simulink model "StampFly_StudentBlocks"  (R2026b)
settings: Solver=VariableStepAuto
undefined symbols (not defined in the file): Bottom, Official
(part 6 of 6)

== stateflow chart StampFly_StudentBlocks/FlightSequence/OfficialTakeoffHover400/SensorProcessing400/AltitudeKalman ==
  note: 高度Kalman：状態=[鉛直速度;高度;加速度バイアス]。400 Hzで最新保持ToFと鉛直加速度を使用。公式resetは内部推定xを保持。
  state Calculate
    en: [height,velocity,bias]=stepFn(alt,az,mode,dt,parkingReset);
    du: [height,velocity,bias]=stepFn(alt,az,mode,dt,parkingReset);
  (default) -> Calculate
  data: alt function_input; az function_input; mode function_input; dt function_input; parkingReset function_input; height function_output; velocity function_output; bias function_output; alt input single; az input single; mode input uint8; dt input single; parkingReset input boolean; height output single; velocity output single; bias output single
  function [height,velocity,bias]=stepFn(alt,az,mode,dt,parkingReset):
    | function [height,velocity,bias]=stepFn(alt,az,mode,dt,parkingReset)
    | % 日本語の説明はブロック注釈とDescriptionを参照。
    | %#codegen
    | persistent State First PreviousMode;
    | if isempty(State)
    | State=kalmanInitial();
    | First=false;
    | PreviousMode=uint8(0);
    | end
    |             if parkingReset,[~,State]=kalmanStep(single(0),single(0),dt,true,State);end
    |             if mode==3 && mode~=PreviousMode,First=false;end
    |             if mode>1
    |                 if First,[~,State]=kalmanStep(alt,az,dt,false,State);else,First=true;end
    |             end
    |             velocity=State.output(1);height=State.output(2);bias=State.output(3);PreviousMode=mode;
    | end
    | 
    | function [y,s] = kalmanStep(z,acc,h,resetState,s)
    | %KALMANSTEP Direct translation of Alt_kalman::update, state [v;z;bias].
    | % Preserve reset(): covariance and public output reset, private x is retained.
    | %#codegen
    | if resetState
    |     s.P = single(100)*eye(3,'single'); s.output(:) = single(0);
    | else
    |     p=s.P; b=single(-0.01); f=single(1)+h*b;
    |     xp=[s.x(1)+(acc-s.x(3))*h;s.x(2)+s.x(1)*h;s.x(3)*f];
    |     pp=zeros(3,3,'single');
    |     pp(1,1)=p(1,1)-h*(p(3,1)+p(1,3))+h*h*p(3,3)+h*h*single(0.01);
    |     pp(1,2)=h*(p(1,1)-p(3,2))-h*h*p(3,1)+p(1,2);
    |     pp(1,3)=f*(p(1,3)-h*p(3,3));
    |     pp(2,1)=h*(p(1,1)-p(2,3))-h*h*p(1,3)+p(2,1);
    |     pp(2,2)=h*h*p(1,1)+h*(p(2,1)+p(1,2))+p(2,2);
    |     pp(2,3)=f*(p(2,3)+h*p(1,3));
    |     pp(3,1)=f*(p(3,1)-h*p(3,3));
    |     pp(3,2)=f*(p(3,2)+h*p(3,1));
    |     pp(3,3)=f*f*p(3,3)+h*h;
    |     k=[pp(1,2);pp(2,2);pp(3,2)]/(pp(2,2)+single(0.004*0.004));
    |     e=z-xp(2); s.x=xp+k*e; s.output=s.x;
    |     s.P(1,:)=pp(1,:)-k(1)*pp(2,:);
    |     s.P(2,:)=pp(2,:)*(single(1)-k(2));
    |     s.P(3,:)=-k(3)*pp(2,:)+pp(3,:);
    | end
    | y=s.output;
    | end
    | 
    | function s = kalmanInitial()
    | %#codegen
    | s = struct('x',zeros(3,1,'single'),'P',single(100)*eye(3,'single'), ...
    |     'output',zeros(3,1,'single'));
    | end

== stateflow chart StampFly_StudentBlocks/FlightSequence/OfficialTakeoffHover400/SensorProcessing400/IMUAxisConversion ==
  note: IMU軸変換：センサーX/Yを入れ替えZの符号を反転。公式の加速度単位gを保持します。
  state Calculate
    en: [a,g]=stepFn(accelMps2,gyroRps);
    du: [a,g]=stepFn(accelMps2,gyroRps);
  (default) -> Calculate
  data: accelMps2 function_input; gyroRps function_input; a function_output; g function_output; accelMps2 input single; gyroRps input single; a output single; g output single
  function [a,g]=stepFn(accelMps2,gyroRps):
    | function [a,g]=stepFn(accelMps2,gyroRps)
    | % 日本語の説明はブロック注釈とDescriptionを参照。
    | %#codegen
    |             a=accelMps2([2 1 3])/single(9.80665);a(3)=-a(3);
    |             g=gyroRps([2 1 3]);g(3)=-g(3);
    | end

== stateflow chart StampFly_StudentBlocks/FlightSequence/OfficialTakeoffHover400/SensorProcessing400/IMUBiasCalibration ==
  note: 800周期の平均校正：ジャイロXYZと加速度Zのオフセットを平均します。400 Hzなので公称2秒です。
  state Calculate
    en: [offset,count]=stepFn(a,g,mode);
    du: [offset,count]=stepFn(a,g,mode);
  (default) -> Calculate
  data: a function_input; g function_input; mode function_input; offset function_output; count function_output; a input single; g input single; mode input uint8; offset output single; count output uint16
  function [offset,count]=stepFn(a,g,mode):
    | function [offset,count]=stepFn(a,g,mode)
    | % 日本語の説明はブロック注釈とDescriptionを参照。
    | %#codegen
    | persistent Offset Count;
    | if isempty(Offset)
    | Offset=zeros(4,1,'single');
    | Count=uint16(0);
    | end
    |             if mode==0,Offset(:)=single(0);Count=uint16(0);
    |             elseif mode==1 && Count<uint16(800)
    |                 n=single(Count);Offset=(n*Offset+[g;a(3)])/(n+single(1));Count=Count+uint16(1);
    |             end
    |             offset=Offset;count=Count;
    | end

== stateflow chart StampFly_StudentBlocks/FlightSequence/OfficialTakeoffHover400/SensorProcessing400/IMUFiltering ==
  note: IMUフィルター：加速度とジャイロは時定数3 ms、鉛直差分は100 ms。PARKING移行で状態をリセット。
  state Calculate
    en: [af,gf,azd]=stepFn(a,g,offset,mode,dt);
    du: [af,gf,azd]=stepFn(a,g,offset,mode,dt);
  (default) -> Calculate
  data: a function_input; g function_input; offset function_input; mode function_input; dt function_input; af function_output; gf function_output; azd function_output; a input single; g input single; offset input single; mode input uint8; dt input single; af output single; gf output single; azd output single
  function [af,gf,azd]=stepFn(a,g,offset,mode,dt):
    | function [af,gf,azd]=stepFn(a,g,offset,mode,dt)
    | % 日本語の説明はブロック注釈とDescriptionを参照。
    | %#codegen
    | persistent Filter Accel Gyro Azd PreviousMode;
    | if isempty(Filter)
    | Filter=zeros(7,1,'single');
    | Accel=zeros(3,1,'single');
    | Gyro=zeros(3,1,'single');
    | Azd=single(0);
    | PreviousMode=uint8(0);
    | end
    |             if mode==3 && mode~=PreviousMode,Filter(:)=single(0);end
    |             if mode>1
    |                 for j=1:3
    |                     Filter(j)=filterStep(a(j),dt,single(0.003),Filter(j));
    |                     Filter(j+3)=filterStep(g(j)-offset(j),dt,single(0.003),Filter(j+3));
    |                 end
    |                 Filter(7)=filterStep(a(3)-offset(4),dt,single(0.1),Filter(7));
    |                 Accel=Filter(1:3);Gyro=Filter(4:6);Azd=Filter(7);
    |             end
    |             af=Accel;gf=Gyro;azd=Azd;PreviousMode=mode;
    | end
    | 
    | function s = filterStep(u,h,T,s)
    | %FILTERSTEP Exact Filter::update, including operation ordering.
    | %#codegen
    | s = s*T/(T+h) + u*h/(T+h);
    | end

== stateflow chart StampFly_StudentBlocks/FlightSequence/OfficialTakeoffHover400/SensorProcessing400/MadgwickAttitude ==
  note: Madgwick姿勢推定：400 Hz、β=0.1。公式の高速逆平方根、軸の対応、Yaw+180°を保持。数式はこのChart内にあります。
  state Calculate
    en: [a,q]=stepFn(rates,accel,mode,reset);
    du: [a,q]=stepFn(rates,accel,mode,reset);
  (default) -> Calculate
  data: arg_rates function_input; arg_accel function_input; arg_mode function_input; arg_reset function_input; arg_a function_output; arg_q function_output; rates input single; accel input single; mode input uint8; reset input boolean; a output single; q output single
  function [arg_a,arg_q]=stepFn(arg_rates,arg_accel,arg_mode,arg_reset):
    | function [arg_a,arg_q]=stepFn(arg_rates,arg_accel,arg_mode,arg_reset)
    | % 日本語の説明はブロック注釈とDescriptionを参照。
    | %#codegen
    | persistent Q Angles;
    | if isempty(Q)
    | Q=single([1;0;0;0]);
    | Angles=zeros(3,1,'single');
    | end
    |             if arg_reset,Q=single([1;0;0;0]);end
    |             if arg_mode>1,[Angles,Q]=madgwickStep(arg_rates,arg_accel,Q,false);end
    |             arg_a=Angles;arg_q=Q;
    | end
    | 
    | function [attitude,arg_q] = madgwickStep(arg_rates,arg_accel,arg_q,arg_reset)
    | %MADGWICKSTEP Official updateIMU with body-axis conventions and invSqrt.
    | % Rates rad/s and arg_accel g in official body frame [forward;left;down].
    | % Madgwick is fixed 400 Hz even though other official filters use measured dt.
    | % Translation of lib/MdgwickAHRS/MadgwickAHRS.cpp; original license retained.
    | %#codegen
    | if arg_reset, arg_q=single([1;0;0;0]); end
    | q0=arg_q(1);q1=arg_q(2);q2=arg_q(3);q3=arg_q(4);
    | % Retain original rad->deg->rad conversion coefficients, including rounding.
    | g=arg_rates([2 1 3])*single(180/pi);g(3)=-g(3);
    | g=g*single(0.0174533);gx=g(1);gy=g(2);gz=g(3);
    | arg_a=arg_accel([2 1 3]);arg_a(3)=-arg_a(3);ax=arg_a(1);ay=arg_a(2);az=arg_a(3);
    | dq=single(0.5)*[-q1*gx-q2*gy-q3*gz; q0*gx+q2*gz-q3*gy; ...
    |     q0*gy-q1*gz+q3*gx; q0*gz+q1*gy-q2*gx];
    | if ax~=0 || ay~=0 || az~=0
    |     reciprocal=fastInvSqrt(ax*ax+ay*ay+az*az);
    |     ax=ax*reciprocal;ay=ay*reciprocal;az=az*reciprocal;
    |     q02=q0*q0;q12=q1*q1;q22=q2*q2;q32=q3*q3;
    |     q0x2=single(2)*q0;q1x2=single(2)*q1;q2x2=single(2)*q2;q3x2=single(2)*q3;
    |     q0x4=single(4)*q0;q1x4=single(4)*q1;q2x4=single(4)*q2;
    |     q1x8=single(8)*q1;q2x8=single(8)*q2;
    |     gradient=[q0x4*q22+q2x2*ax+q0x4*q12-q1x2*ay; ...
    |         q1x4*q32-q3x2*ax+single(4)*q02*q1-q0x2*ay-q1x4+q1x8*q12+q1x8*q22+q1x4*az; ...
    |         single(4)*q02*q2+q0x2*ax+q2x4*q32-q3x2*ay-q2x4+q2x8*q12+q2x8*q22+q2x4*az; ...
    |         single(4)*q12*q3-q1x2*ax+single(4)*q22*q3-q2x2*ay];
    |     reciprocal=fastInvSqrt(gradient(1)*gradient(1)+gradient(2)*gradient(2)+gradient(3)*gradient(3)+gradient(4)*gradient(4));
    |     gradient=gradient*reciprocal;
    |     dq=dq-single(0.1)*gradient;
    | end
    | arg_q=arg_q+dq*single(1/400);
    | reciprocal=fastInvSqrt(arg_q(1)*arg_q(1)+arg_q(2)*arg_q(2)+arg_q(3)*arg_q(3)+arg_q(4)*arg_q(4));arg_q=arg_q*reciprocal;
    | roll=atan2(arg_q(1)*arg_q(2)+arg_q(3)*arg_q(4),single(0.5)-arg_q(2)*arg_q(2)-arg_q(3)*arg_q(3));
    | pitch=asin(-single(2)*(arg_q(2)*arg_q(4)-arg_q(1)*arg_q(3)));
    | yaw=atan2(arg_q(2)*arg_q(3)+arg_q(1)*arg_q(4),single(0.5)-arg_q(3)*arg_q(3)-arg_q(4)*arg_q(4));
    | % Original getYaw adds 180 degrees; do not hide this offset.
    | attitude=[pitch*single(57.29578);roll*single(57.29578); ...
    |     -(yaw*single(57.29578)+single(180))]*single(pi/180);
    | end
    | 
    | function y=fastInvSqrt(x)
    | i=typecast(x,'uint32');i=uint32(hex2dec('5f3759df'))-bitshift(i,-1);
    | y=typecast(i,'single');half=single(0.5)*x;
    | y=y*(single(1.5)-half*y*y);y=y*(single(1.5)-half*y*y);
    | end

== stateflow chart StampFly_StudentBlocks/FlightSequence/OfficialTakeoffHover400/SensorProcessing400/SensorDiagnosticPack ==
  state Calculate
    en: [diag]=stepFn(az,bias,alt,offset,count);
    du: [diag]=stepFn(az,bias,alt,offset,count);
  (default) -> Calculate
  data: az function_input; bias function_input; alt function_input; offset function_input; count function_input; diag function_output; az input single; bias input single; alt input single; offset input single; count input uint16; diag output single
  function diag =stepFn(az,bias,alt,offset,count):
    | function diag =stepFn(az,bias,alt,offset,count)
    | % 日本語の説明はブロック注釈とDescriptionを参照。
    | %#codegen
    |             diag=[az;bias;alt;offset;single(count)];
    | end

== stateflow chart StampFly_StudentBlocks/Estimation/IMUFiltering ==
  note: IMUフィルター：加速度とジャイロは時定数3 ms、鉛直差分は100 ms。PARKING移行で状態をリセット。
  state Calculate
    en: [af,gf,azd]=stepFn(a,g,offset,mode,dt);
    du: [af,gf,azd]=stepFn(a,g,offset,mode,dt);
  (default) -> Calculate
  data: a function_input; g function_input; offset function_input; mode function_input; dt function_input; af function_output; gf function_output; azd function_output; a input single; g input single; offset input single; mode input uint8; dt input single; af output single; gf output single; azd output single
  function [af,gf,azd]=stepFn(a,g,offset,mode,dt):
    | function [af,gf,azd]=stepFn(a,g,offset,mode,dt)
    | % 日本語の説明はブロック注釈とDescriptionを参照。
    | %#codegen
    | persistent Filter Accel Gyro Azd PreviousMode;
    | if isempty(Filter)
    | Filter=zeros(7,1,'single');
    | Accel=zeros(3,1,'single');
    | Gyro=zeros(3,1,'single');
    | Azd=single(0);
    | PreviousMode=uint8(0);
    | end
    |             if mode==3 && mode~=PreviousMode,Filter(:)=single(0);end
    |             if mode>1
    |                 for j=1:3
    |                     Filter(j)=filterStep(a(j),dt,single(0.003),Filter(j));
    |                     Filter(j+3)=filterStep(g(j)-offset(j),dt,single(0.003),Filter(j+3));
    |                 end
    |                 Filter(7)=filterStep(a(3)-offset(4),dt,single(0.1),Filter(7));
    |                 Accel=Filter(1:3);Gyro=Filter(4:6);Azd=Filter(7);
    |             end
    |             af=Accel;gf=Gyro;azd=Azd;PreviousMode=mode;
    | end
    | 
    | function s = filterStep(u,h,T,s)
    | %FILTERSTEP Exact Filter::update, including operation ordering.
    | %#codegen
    | s = s*T/(T+h) + u*h/(T+h);
    | end

== stateflow chart StampFly_StudentBlocks/FlightSequence/OfficialTakeoffHover400/SensorProcessing400/SensorFlags ==
  note: フラグ判定：OverG、距離無効/高度上限、低電圧100回。PID制御や状態遷移で使います。
  state Calculate
    en: [flags]=stepFn(accel,azd,voltage,mode,altFlag,height,rawRange,dt,parkingReset,flipFlag);
    du: [flags]=stepFn(accel,azd,voltage,mode,altFlag,height,rawRange,dt,parkingReset,flipFlag);
  (default) -> Calculate
  data: arg_accel function_input; arg_azd function_input; arg_voltage function_input; arg_mode function_input; arg_altFlag function_input; arg_height function_input; arg_rawRange function_input; arg_dt function_input; arg_parkingReset function_input; arg_flags function_output; arg_flipFlag function_input; accel input single; azd input single; voltage input single; mode input uint8; altFlag input uint8; height input single; rawRange input int16; dt input single; parkingReset input boolean; flags output uint8; flipFlag input uint8
  function arg_flags =stepFn(arg_accel,arg_azd,arg_voltage,arg_mode,arg_altFlag,arg_height,arg_rawRange,arg_dt,arg_parkingReset,arg_flipFlag):
    | function arg_flags =stepFn(arg_accel,arg_azd,arg_voltage,arg_mode,arg_altFlag,arg_height,arg_rawRange,arg_dt,arg_parkingReset,arg_flipFlag)
    | % 日本語の説明はブロック注釈とDescriptionを参照。
    | %#codegen
    | persistent Norm Voltage OverG RangeFlag LowVoltage PreviousMode;
    | if isempty(Norm)
    | Norm=single(0);
    | Voltage=single(0);
    | OverG=uint8(0);
    | RangeFlag=uint8(0);
    | LowVoltage=uint8(0);
    | PreviousMode=uint8(0);
    | end
    |             if arg_parkingReset,OverG=uint8(0);RangeFlag=uint8(0);end
    |             if arg_mode==3 && arg_mode~=PreviousMode,Norm=single(0);end
    |             if arg_mode>1
    |                 if (arg_height>single(2) && arg_altFlag~=0 && arg_flipFlag==0) || arg_rawRange==0,RangeFlag=min(RangeFlag+uint8(1),uint8(20));else,RangeFlag=uint8(0);end
    |             end
    |             normA=sqrt(arg_accel(1)*arg_accel(1)+arg_accel(2)*arg_accel(2)+arg_azd*arg_azd);
    |             Norm=filterStep(normA,arg_dt,single(.005),Norm);
    |             if Norm>single(2),OverG=uint8(1);end
    |             Voltage=filterStep(arg_voltage,arg_dt,single(.005),Voltage);
    |             if LowVoltage~=uint8(100)
    |                 if Voltage<single(3.34),LowVoltage=LowVoltage+uint8(1);else,LowVoltage=uint8(0);end
    |                 LowVoltage=min(LowVoltage,uint8(100));
    |             end
    |             arg_flags=[OverG;RangeFlag;LowVoltage];PreviousMode=arg_mode;
    | end
    | 
    | function s = filterStep(u,h,T,s)
    | %FILTERSTEP Exact Filter::update, including operation ordering.
    | %#codegen
    | s = s*T/(T+h) + u*h/(T+h);
    | end

== stateflow chart StampFly_StudentBlocks/FlightSequence/OfficialTakeoffHover400/SensorProcessing400/ToFHoldOutlierFilter ==
  note: ToF処理：新データ時に距離を更新。20 mm以下は保持、500 mmを超える飛びは最大2回補外。5 msフィルター。
  state Calculate
    en: [alt,raw]=stepFn(mm,fresh,mode,dt);
    du: [alt,raw]=stepFn(mm,fresh,mode,dt);
  (default) -> Calculate
  data: mm function_input; fresh function_input; mode function_input; dt function_input; alt function_output; raw function_output; mm input int16; fresh input uint8; mode input uint8; dt input single; alt output single; raw output int16
  function [alt,raw]=stepFn(mm,fresh,mode,dt):
    | function [alt,raw]=stepFn(mm,fresh,mode,dt)
    | % 日本語の説明はブロック注釈とDescriptionを参照。
    | %#codegen
    | persistent History Range Raw Outlier Alt PreviousMode;
    | if isempty(History)
    | History=zeros(4,1,'int16');
    | Range=int16(0);
    | Raw=int16(0);
    | Outlier=uint8(0);
    | Alt=single(0);
    | PreviousMode=uint8(0);
    | end
    |             if mode==3 && mode~=PreviousMode,History(:)=int16(0);Alt=single(0);end
    |             if mode>1
    |                 if fresh~=0
    |                     Raw=mm;if mm>int16(20),Range=mm;end
    |                     delta=int32(Range)-int32(History(2));
    |                     if abs(delta)>int32(500) && Outlier<uint8(2)
    |                         extrap=int32(History(2))+idivide(int32(History(2))-int32(History(4)),int32(2),'fix');
    |                         Range=int16(extrap);Outlier=Outlier+uint8(1);
    |                     else
    |                         Outlier=uint8(0);History(4)=History(3);History(3)=History(2);History(2)=Range;
    |                     end
    |                 end
    |                 Alt=filterStep(single(double(Range)/1000),dt,single(0.005),Alt);
    |             end
    |             alt=Alt;raw=Raw;PreviousMode=mode;
    | end
    | 
    | function s = filterStep(u,h,T,s)
    | %FILTERSTEP Exact Filter::update, including operation ordering.
    | %#codegen
    | s = s*T/(T+h) + u*h/(T+h);
    | end

== stateflow chart StampFly_StudentBlocks/FlightSequence/OfficialTakeoffHover400/SensorProcessing400/VerticalAcceleration ==
  note: 鉛直加速度：校正後AccelZ差分を反転して100 msフィルター。公式に合わせ単位gのまま高度Kalmanへ入力。
  state Calculate
    en: [az]=stepFn(azd,mode,dt);
    du: [az]=stepFn(azd,mode,dt);
  (default) -> Calculate
  data: azd function_input; mode function_input; dt function_input; az function_output; azd input single; mode input uint8; dt input single; az output single
  function az =stepFn(azd,mode,dt):
    | function az =stepFn(azd,mode,dt)
    | % 日本語の説明はブロック注釈とDescriptionを参照。
    | %#codegen
    | persistent Az PreviousMode;
    | if isempty(Az)
    | Az=single(0);
    | PreviousMode=uint8(0);
    | end
    |             if mode==3 && mode~=PreviousMode,Az=single(0);end
    |             if mode>1,Az=filterStep(-azd,dt,single(0.1),Az);end
    |             az=Az;PreviousMode=mode;
    | end
    | 
    | function s = filterStep(u,h,T,s)
    | %FILTERSTEP Exact Filter::update, including operation ordering.
    | %#codegen
    | s = s*T/(T+h) + u*h/(T+h);
    | end

== stateflow chart StampFly_StudentBlocks/FlightSequence/OfficialTakeoffHover400/TakeoffHoverControl400/ControlDiagnosticPack ==
  state Calculate
    en: [diag]=stepFn(alt,base,counter,zRef,thrust,angle,rate,rollTorque,pitchTorque,yawTorque,before);
    du: [diag]=stepFn(alt,base,counter,zRef,thrust,angle,rate,rollTorque,pitchTorque,yawTorque,before);
  (default) -> Calculate
  data: alt function_input; base function_input; counter function_input; zRef function_input; thrust function_input; angle function_input; rate function_input; rollTorque function_input; pitchTorque function_input; yawTorque function_input; before function_input; diag function_output; alt input single; base input single; counter input uint16; zRef input single; thrust input single; angle input single; rate input single; rollTorque input single; pitchTorque input single; yawTorque input single; before input single; diag output single
  function diag =stepFn(alt,base,counter,zRef,thrust,angle,rate,rollTorque,pitchTorque,yawTorque,before):
    | function diag =stepFn(alt,base,counter,zRef,thrust,angle,rate,rollTorque,pitchTorque,yawTorque,before)
    | % 日本語の説明はブロック注釈とDescriptionを参照。
    | %#codegen
    |             diag=[alt;base;single(counter);zRef;thrust;angle;rate;rollTorque;pitchTorque;yawTorque;before];
    | end

== stateflow chart StampFly_StudentBlocks/FlightSequence/OfficialTakeoffHover400/TakeoffHoverControl400/ControlEnableReset ==
  note: 実行/リセット判定：推力Dutyが0.1未満ならPIDをリセットし、各ループのEnableを決めます。
  state Calculate
    en: [command,run,reset,altEnable,angleEnable,velEnable,angleReset,flipFlag]=stepFn(raw,manual,auto,mode,controlMode,dt,oldFilter,lastThrust,phase,flipThrust,flipStart,flipDone,finalMode);
    du: [command,run,reset,altEnable,angleEnable,velEnable,angleReset,flipFlag]=stepFn(raw,manual,auto,mode,controlMode,dt,oldFilter,lastThrust,phase,flipThrust,flipStart,flipDone,finalMode);
  (default) -> Calculate
  data: arg_arg_raw function_input; arg_arg_manual function_input; arg_arg_auto function_input; arg_branch function_input; arg_arg_controlMode function_input; arg_arg_dt function_input; arg_arg_oldFilter function_input; arg_arg_lastThrust function_input; arg_arg_command function_output; arg_arg_run function_output; arg_arg_reset function_output; arg_arg_altEnable function_output; arg_arg_angleEnable function_output; arg_arg_velEnable function_output; arg_arg_phase function_input; arg_arg_flipThrust function_input; arg_arg_flipStart function_input; arg_arg_flipDone function_input; arg_arg_mode function_input; arg_arg_angleReset function_output; arg_arg_flipFlag function_output; raw input single; manual input boolean; auto input boolean; mode input uint8; controlMode input single; dt input single; oldFilter input single; lastThrust input single; command output single; run output boolean; reset output boolean; altEnable output boolean; angleEnable output boolean; velEnable output boolean; phase input uint8; flipThrust input single; flipStart input boolean; flipDone input boolean; finalMode input uint8; angleReset output boolean; flipFlag output uint8
  function [arg_arg_command,arg_arg_run,arg_arg_reset,arg_arg_altEnable,arg_arg_angleEnable,arg_arg_velEnable,arg_arg_angleReset,arg_arg_flipFlag]=stepFn(arg_arg_raw,arg_arg_manual,arg_arg_auto,arg_branch,arg_arg_controlMode,arg_arg_dt,arg_arg_oldFilter,arg_arg_lastThrust,arg_arg_phase,arg_arg_flipThrust,arg_arg_flipStart,arg_arg_flipDone,arg_arg_mode):
    | function [arg_arg_command,arg_arg_run,arg_arg_reset,arg_arg_altEnable,arg_arg_angleEnable,arg_arg_velEnable,arg_arg_angleReset,arg_arg_flipFlag]=stepFn(arg_arg_raw,arg_arg_manual,arg_arg_auto,arg_branch,arg_arg_controlMode,arg_arg_dt,arg_arg_oldFilter,arg_arg_lastThrust,arg_arg_phase,arg_arg_flipThrust,arg_arg_flipStart,arg_arg_flipDone,arg_arg_mode)
    | % angle_controlとrate_controlで異なるリセット条件を保持する。
    | %#codegen
    | persistent heldFlip;
    | if isempty(heldFlip),heldFlip=uint8(0);end
    | arg_arg_command=arg_arg_raw;
    | if arg_arg_manual,arg_arg_command=filterStep(arg_arg_raw,arg_arg_dt,single(.01),arg_arg_oldFilter);end
    | if arg_branch==5 || arg_branch==3 || arg_arg_flipDone,arg_arg_command=arg_arg_lastThrust;end
    | if arg_branch==6 && arg_arg_phase>0,arg_arg_command=arg_arg_flipThrust;end
    | active=arg_branch==2 || arg_branch==5 || (arg_branch==6 && ~arg_arg_flipDone);
    | angleCalled=active && (arg_arg_phase==0 || arg_arg_phase==1);
    | arg_arg_angleReset=angleCalled && double(arg_arg_command)/3.7<double(single(.1));
    | arg_arg_flipFlag=heldFlip;
    | if arg_branch==3 || arg_arg_flipDone,arg_arg_flipFlag=uint8(0);end
    | if arg_branch==6 && ~arg_arg_flipDone,arg_arg_flipFlag=arg_arg_phase;end
    | if arg_arg_flipStart,arg_arg_flipFlag=uint8(1);end
    | if arg_arg_angleReset,arg_arg_flipFlag=uint8(0);end
    | arg_arg_reset=active && double(arg_arg_command)/3.7<double(single(.1)) && arg_arg_flipFlag==0;
    | arg_arg_run=active && ~arg_arg_reset;
    | arg_arg_altEnable=angleCalled && ~arg_arg_angleReset && arg_arg_auto;
    | arg_arg_angleEnable=angleCalled && ~arg_arg_angleReset && uint8(arg_arg_controlMode)==0;
    | arg_arg_velEnable=arg_arg_run && ((arg_arg_auto && arg_arg_flipFlag==0) || arg_arg_mode==5);
    | if arg_arg_reset,arg_arg_flipFlag=uint8(0);end
    | heldFlip=arg_arg_flipFlag;
    | end
    | function s=filterStep(u,h,T,s),s=s*T/(T+h)+u*h/(T+h);end

== stateflow chart StampFly_StudentBlocks/FlightSequence/OfficialTakeoffHover400/TakeoffHoverControl400/FinalizeFlightMode ==
  state Calculate
    en: [mode]=stepFn(branch,preMode,height,flipStart,flipDone,overG);
    du: [mode]=stepFn(branch,preMode,height,flipStart,flipDone,overG);
  (default) -> Calculate
  data: arg_branch function_input; arg_preMode function_input; arg_height function_input; arg_flipStart function_input; arg_flipDone function_input; arg_overG function_input; arg_mode function_output; branch input uint8; preMode input uint8; height input single; flipStart input boolean; flipDone input boolean; overG input uint8; mode output uint8
  function arg_mode=stepFn(arg_branch,arg_preMode,arg_height,arg_flipStart,arg_flipDone,arg_overG):
    | function arg_mode=stepFn(arg_branch,arg_preMode,arg_height,arg_flipStart,arg_flipDone,arg_overG)
    | % loop分岐の途中で変わるMode。get_commandは分岐途中でもFlipに変更できる。
    | %#codegen
    | arg_mode=arg_preMode;
    | if arg_branch==5 && arg_height<.1,arg_mode=uint8(3);end
    | if arg_flipStart && (arg_branch==2 || arg_branch==6),arg_mode=uint8(6);end
    | if arg_branch==6 && arg_flipDone,arg_mode=uint8(2);end
    | if (arg_branch==2 || arg_branch==5 || arg_branch==6) && arg_overG==1,arg_mode=uint8(3);end
    | end

== stateflow chart StampFly_StudentBlocks/FlightSequence/OfficialTakeoffHover400/TakeoffHoverControl400/SelectRateReference ==
  state Calculate
    en: [rate]=stepFn(direct,rollPID,pitchPID,angleEnable);
    du: [rate]=stepFn(direct,rollPID,pitchPID,angleEnable);
  (default) -> Calculate
  data: direct function_input; rollPID function_input; pitchPID function_input; angleEnable function_input; rate function_output; direct input single; rollPID input single; pitchPID input single; angleEnable input boolean; rate output single
  function rate =stepFn(direct,rollPID,pitchPID,angleEnable):
    | function rate =stepFn(direct,rollPID,pitchPID,angleEnable)
    | % 日本語の説明はブロック注釈とDescriptionを参照。
    | %#codegen
    |             rate=direct;if angleEnable,rate(1)=rollPID;rate(2)=pitchPID;end
    | end

== stateflow chart StampFly_StudentBlocks/FlightSequence/OfficialTakeoffHover400/TakeoffHoverControl400/SelectVerticalReference ==
  state Calculate
    en: [vRef]=stepFn(zRef,mode,auto,flipFlag);
    du: [vRef]=stepFn(zRef,mode,auto,flipFlag);
  (default) -> Calculate
  data: arg_zRef function_input; arg_mode function_input; arg_vRef function_output; arg_auto function_input; arg_flipFlag function_input; zRef input single; mode input uint8; vRef output single; auto input boolean; flipFlag input uint8
  function arg_vRef=stepFn(arg_zRef,arg_mode,arg_auto,arg_flipFlag):
    | function arg_vRef=stepFn(arg_zRef,arg_mode,arg_auto,arg_flipFlag)
    | % Auto高度補正が優先。公式else-ifの順序を維持。
    | %#codegen
    | arg_vRef=arg_zRef;if ~(arg_auto && arg_flipFlag==0) && arg_mode==5,arg_vRef=single(-.15);end
    | end

== stateflow chart StampFly_StudentBlocks/FlightSequence/OfficialTakeoffHover400/TakeoffHoverControl400/StickToAngleRate ==
  note: スティック→目標：Stabilizeは角度±30°、Sportは角速度カーブ。中立位置は低推力時に保存。Yawは角速度指令。
  state Calculate
    en: [angle,directRate,resetError]=stepFn(stick,mode,run,reset,phase,flipRate,angleReset,lastRate,flipDone,controlMode);
    du: [angle,directRate,resetError]=stepFn(stick,mode,run,reset,phase,flipRate,angleReset,lastRate,flipDone,controlMode);
  (default) -> Calculate
  data: arg_arg_stick function_input; arg_branch function_input; arg_arg_run function_input; arg_arg_reset function_input; arg_arg_angle function_output; arg_arg_directRate function_output; arg_arg_resetError function_output; arg_arg_phase function_input; arg_arg_flipRate function_input; arg_arg_angleReset function_input; arg_arg_lastRate function_input; arg_arg_flipDone function_input; arg_arg_controlMode function_input; stick input single; mode input uint8; run input boolean; reset input boolean; angle output single; directRate output single; resetError output single; phase input uint8; flipRate input single; angleReset input boolean; lastRate input single; flipDone input boolean; controlMode input single
  function [arg_arg_angle,arg_arg_directRate,arg_arg_resetError]=stepFn(arg_arg_stick,arg_branch,arg_arg_run,arg_arg_reset,arg_arg_phase,arg_arg_flipRate,arg_arg_angleReset,arg_arg_lastRate,arg_arg_flipDone,arg_arg_controlMode):
    | function [arg_arg_angle,arg_arg_directRate,arg_arg_resetError]=stepFn(arg_arg_stick,arg_branch,arg_arg_run,arg_arg_reset,arg_arg_phase,arg_arg_flipRate,arg_arg_angleReset,arg_arg_lastRate,arg_arg_flipDone,arg_arg_controlMode)
    | % command、角度目標、中立点を別々に保持。Sportは角度commandを更新しない。
    | %#codegen
    | persistent Angle Centers AngleCmd YawCmd;
    | if isempty(Angle),Angle=zeros(2,1,'single');Centers=zeros(3,1,'single');AngleCmd=zeros(2,1,'single');YawCmd=single(0);end
    | arg_arg_directRate=arg_arg_lastRate;arg_arg_resetError=Angle;
    | commandCalled=arg_branch==2 || arg_branch==5 || (arg_branch==6 && arg_arg_phase==0 && ~arg_arg_flipDone);
    | if commandCalled
    |  if uint8(arg_arg_controlMode)==0 || arg_branch==5,AngleCmd=min(max(single(.4*double(arg_arg_stick(1:2))),single(-1)),single(1));end
    |  YawCmd=min(max(arg_arg_stick(3),single(-1)),single(1));
    |  arg_arg_directRate(3)=single(2*pi*double(YawCmd-Centers(3)));
    |  if uint8(arg_arg_controlMode)==1,arg_arg_directRate(1)=rateCommand(arg_arg_stick(1));arg_arg_directRate(2)=rateCommand(arg_arg_stick(2));end
    | elseif arg_branch==6 && arg_arg_phase==1,AngleCmd(:)=single(0);
    | end
    | if arg_arg_angleReset,Centers(1:2)=AngleCmd;end
    | if arg_arg_reset,Centers(3)=YawCmd;end
    | if arg_arg_run && (arg_arg_phase==0 || arg_arg_phase==1) && uint8(arg_arg_controlMode)==0
    |  limit=single(30*pi/180);Angle=min(max(single(.5*pi*double(AngleCmd-Centers(1:2))),-limit),limit);
    | end
    | if arg_branch==6 && arg_arg_phase>=2,arg_arg_directRate(1)=arg_arg_flipRate;arg_arg_directRate(2)=single(0);end
    | if arg_branch==3,arg_arg_directRate(1)=single(0);end
    | if arg_arg_reset,arg_arg_directRate(:)=single(0);end
    | arg_arg_angle=Angle;
    | end
    | function y=rateCommand(x)
    | x=min(max(x,single(-1)),single(1));a=abs(x);t=a*(a*a*a*a*a*single(.5)+a*single(.5));
    | y=single(pi/180)*((single(1600)-single(70))*t+single(70)*a);if x<0,y=-y;end
    | end

== stateflow chart StampFly_StudentBlocks/Estimation/IMUAxisConversion ==
  note: IMU軸変換：センサーX/Yを入れ替えZの符号を反転。公式の加速度単位gを保持します。
  state Calculate
    en: [a,g]=stepFn(accelMps2,gyroRps);
    du: [a,g]=stepFn(accelMps2,gyroRps);
  (default) -> Calculate
  data: accelMps2 function_input; gyroRps function_input; a function_output; g function_output; accelMps2 input single; gyroRps input single; a output single; g output single
  function [a,g]=stepFn(accelMps2,gyroRps):
    | function [a,g]=stepFn(accelMps2,gyroRps)
    | % 日本語の説明はブロック注釈とDescriptionを参照。
    | %#codegen
    |             a=accelMps2([2 1 3])/single(9.80665);a(3)=-a(3);
    |             g=gyroRps([2 1 3]);g(3)=-g(3);
    | end

== stateflow chart StampFly_StudentBlocks/FlightSequence/OfficialTakeoffHover400/TakeoffHoverControl400/TakeoffLandingCommand ==
  note: 離陸/着陸の指令：離陸カウンター0〜1000、初期高度0.5 m、上下スティックで0.05〜1.8 m。電圧トリム=-0.2448V+1.5892。
  state Calculate
    en: [alt,base,counter,raw,auto,manual,controlMode]=stepFn(stick,height,voltage,rangeFlag,mode,phase,flipDone);
    du: [alt,base,counter,raw,auto,manual,controlMode]=stepFn(stick,height,voltage,rangeFlag,mode,phase,flipDone);
  (default) -> Calculate
  data: arg_arg_stick function_input; arg_arg_height function_input; arg_arg_voltage function_input; arg_arg_rangeFlag function_input; arg_branch function_input; arg_arg_alt function_output; arg_arg_base function_output; arg_arg_counter function_output; arg_arg_raw function_output; arg_arg_auto function_output; arg_arg_manual function_output; arg_arg_phase function_input; arg_arg_flipDone function_input; arg_arg_controlMode function_output; stick input single; height input single; voltage input single; rangeFlag input uint8; mode input uint8; alt output single; base output single; counter output uint16; raw output single; auto output boolean; manual output boolean; phase input uint8; flipDone input boolean; controlMode output single
  function [arg_arg_alt,arg_arg_base,arg_arg_counter,arg_arg_raw,arg_arg_auto,arg_arg_manual,arg_arg_controlMode]=stepFn(arg_arg_stick,arg_arg_height,arg_arg_voltage,arg_arg_rangeFlag,arg_branch,arg_arg_phase,arg_arg_flipDone):
    | function [arg_arg_alt,arg_arg_base,arg_arg_counter,arg_arg_raw,arg_arg_auto,arg_arg_manual,arg_arg_controlMode]=stepFn(arg_arg_stick,arg_arg_height,arg_arg_voltage,arg_arg_rangeFlag,arg_branch,arg_arg_phase,arg_arg_flipDone)
    | % 公式get_command/auto_landing。Alt_flagはManual切替時にも保持される。
    | %#codegen
    | persistent Alt Base Counter RangeOld Landing History AltFlag ControlMode;
    | if isempty(Alt)
    |  Alt=single(.5);Base=single(0);Counter=uint16(0);RangeOld=uint8(0);
    |  Landing=false;History=zeros(10,1,'single');AltFlag=false;ControlMode=uint8(0);
    | end
    | arg_arg_raw=single(0);arg_arg_manual=false;
    | if arg_branch==3
    |  Base=single(0);Alt=single(.5);Counter=uint16(0);Landing=false;AltFlag=false;
    | elseif arg_branch==2 || (arg_branch==6 && arg_arg_phase==0 && ~arg_arg_flipDone)
    |  ControlMode=uint8(arg_arg_stick(5));
    |  if uint8(arg_arg_stick(6))==4
    |   AltFlag=true;
    |   if Counter<500
    |    Base=min(single(Counter)/single(1000),trim(single(3.8)));Counter=Counter+uint16(1);
    |   elseif Counter<1000
    |    Base=min(single(Counter)/single(1000),trim(arg_arg_voltage));Counter=Counter+uint16(1);
    |   else,Base=trim(arg_arg_voltage);end
    |   th=arg_arg_stick(4);if th>-.2 && th<.2,th=single(0);end
    |   Alt=min(max(single(double(Alt)+double(th)*.001),single(.05)),single(1.8));
    |   if arg_arg_rangeFlag>RangeOld || arg_arg_rangeFlag==20,Base=Base-single(.02);RangeOld=arg_arg_rangeFlag;end
    |   arg_arg_raw=single(double(Base)*3.7);
    |  else
    |   arg_arg_manual=true;th=min(max(arg_arg_stick(4),single(0)),single(1));
    |   if th>-.2 && th<.2,th=single(0);end
    |   arg_arg_raw=single((.00413+double(single(3.3)*th-single(5.44)*th*th+single(3.13)*th*th*th))*3.7);
    |  end
    | elseif arg_branch==5
    |  AltFlag=false;
    |  if ~Landing,Landing=true;History(:)=arg_arg_height;Base=trim(arg_arg_voltage);end
    |  if History(10)>=arg_arg_height,Base=single(double(Base)*.9999);end
    |  if arg_arg_height<.15,Base=single(double(Base)*.999);end
    |  if arg_arg_height<.1,Landing=false;end
    |  for j=2:10,History(j)=History(j-1);end
    |  History(1)=arg_arg_height;
    | end
    | arg_arg_alt=Alt;arg_arg_base=Base;arg_arg_counter=Counter;arg_arg_auto=AltFlag;arg_arg_controlMode=single(ControlMode);
    | end
    | function y=trim(v),y=-single(.2448)*v+single(1.5892);end

== stateflow chart StampFly_StudentBlocks/FlightSequence/OfficialTakeoffHover400/TakeoffHoverControl400/ThrustCorrectionLimits ==
  note: 鉛直速度PID補正から推力を生成。10 msフィルター後、Auto高度では基準推力の0.85〜1.15倍に制限。
  state Calculate
    en: [thrust,filter,last]=stepFn(command,correction,base,auto,manual,velEnable,mode,dt,oldFilter,lastThrust,flipFlag);
    du: [thrust,filter,last]=stepFn(command,correction,base,auto,manual,velEnable,mode,dt,oldFilter,lastThrust,flipFlag);
  (default) -> Calculate
  data: arg_arg_command function_input; arg_arg_correction function_input; arg_arg_base function_input; arg_arg_auto function_input; arg_arg_manual function_input; arg_arg_velEnable function_input; arg_branch function_input; arg_arg_dt function_input; arg_arg_oldFilter function_input; arg_arg_lastThrust function_input; arg_arg_thrust function_output; arg_arg_filter function_output; arg_arg_last function_output; arg_arg_flipFlag function_input; command input single; correction input single; base input single; auto input boolean; manual input boolean; velEnable input boolean; mode input uint8; dt input single; oldFilter input single; lastThrust input single; thrust output single; filter output single; last output single; flipFlag input uint8
  function [arg_arg_thrust,arg_arg_filter,arg_arg_last]=stepFn(arg_arg_command,arg_arg_correction,arg_arg_base,arg_arg_auto,arg_arg_manual,arg_arg_velEnable,arg_branch,arg_arg_dt,arg_arg_oldFilter,arg_arg_lastThrust,arg_arg_flipFlag):
    | function [arg_arg_thrust,arg_arg_filter,arg_arg_last]=stepFn(arg_arg_command,arg_arg_correction,arg_arg_base,arg_arg_auto,arg_arg_manual,arg_arg_velEnable,arg_branch,arg_arg_dt,arg_arg_oldFilter,arg_arg_lastThrust,arg_arg_flipFlag)
    | % rate_control: Auto補正がLanding補正より優先。Flip中はAuto補正を停止。
    | %#codegen
    | arg_arg_thrust=arg_arg_command;arg_arg_filter=arg_arg_oldFilter;
    | if arg_branch==3,arg_arg_filter=single(0);elseif arg_arg_manual,arg_arg_filter=arg_arg_command;end
    | if arg_arg_velEnable
    |  arg_arg_filter=filterStep(single(double(arg_arg_base+arg_arg_correction)*3.7),arg_arg_dt,single(.01),arg_arg_filter);arg_arg_thrust=arg_arg_filter;
    |  if arg_arg_auto && arg_arg_flipFlag==0
    |   if double(arg_arg_thrust)/3.7>double(single(arg_arg_base*single(1.15))),arg_arg_thrust=single(3.7*double(arg_arg_base)*double(single(1.15)));end
    |   if double(arg_arg_thrust)/3.7<double(single(arg_arg_base*single(.85))),arg_arg_thrust=single(3.7*double(arg_arg_base)*double(single(.85)));end
    |  end
    | end
    | if arg_branch==3,arg_arg_thrust=arg_arg_lastThrust;arg_arg_last=arg_arg_lastThrust;else,arg_arg_last=arg_arg_thrust;end
    | end
    | function s=filterStep(u,h,T,s),s=s*T/(T+h)+u*h/(T+h);end

== stateflow chart StampFly_StudentBlocks/Controllers/StickToAngleRate ==
  note: スティック→目標：Stabilizeは角度±30°、Sportは角速度カーブ。中立位置は低推力時に保存。Yawは角速度指令。
  state Calculate
    en: [angle,directRate,resetError]=stepFn(stick,mode,run,reset,phase,flipRate,angleReset,lastRate,flipDone,controlMode);
    du: [angle,directRate,resetError]=stepFn(stick,mode,run,reset,phase,flipRate,angleReset,lastRate,flipDone,controlMode);
  (default) -> Calculate
  data: arg_arg_stick function_input; arg_branch function_input; arg_arg_run function_input; arg_arg_reset function_input; arg_arg_angle function_output; arg_arg_directRate function_output; arg_arg_resetError function_output; arg_arg_phase function_input; arg_arg_flipRate function_input; arg_arg_angleReset function_input; arg_arg_lastRate function_input; arg_arg_flipDone function_input; arg_arg_controlMode function_input; stick input single; mode input uint8; run input boolean; reset input boolean; angle output single; directRate output single; resetError output single; phase input uint8; flipRate input single; angleReset input boolean; lastRate input single; flipDone input boolean; controlMode input single
  function [arg_arg_angle,arg_arg_directRate,arg_arg_resetError]=stepFn(arg_arg_stick,arg_branch,arg_arg_run,arg_arg_reset,arg_arg_phase,arg_arg_flipRate,arg_arg_angleReset,arg_arg_lastRate,arg_arg_flipDone,arg_arg_controlMode):
    | function [arg_arg_angle,arg_arg_directRate,arg_arg_resetError]=stepFn(arg_arg_stick,arg_branch,arg_arg_run,arg_arg_reset,arg_arg_phase,arg_arg_flipRate,arg_arg_angleReset,arg_arg_lastRate,arg_arg_flipDone,arg_arg_controlMode)
    | % command、角度目標、中立点を別々に保持。Sportは角度commandを更新しない。
    | %#codegen
    | persistent Angle Centers AngleCmd YawCmd;
    | if isempty(Angle),Angle=zeros(2,1,'single');Centers=zeros(3,1,'single');AngleCmd=zeros(2,1,'single');YawCmd=single(0);end
    | arg_arg_directRate=arg_arg_lastRate;arg_arg_resetError=Angle;
    | commandCalled=arg_branch==2 || arg_branch==5 || (arg_branch==6 && arg_arg_phase==0 && ~arg_arg_flipDone);
    | if commandCalled
    |  if uint8(arg_arg_controlMode)==0 || arg_branch==5,AngleCmd=min(max(single(.4*double(arg_arg_stick(1:2))),single(-1)),single(1));end
    |  YawCmd=min(max(arg_arg_stick(3),single(-1)),single(1));
    |  arg_arg_directRate(3)=single(2*pi*double(YawCmd-Centers(3)));
    |  if uint8(arg_arg_controlMode)==1,arg_arg_directRate(1)=rateCommand(arg_arg_stick(1));arg_arg_directRate(2)=rateCommand(arg_arg_stick(2));end
    | elseif arg_branch==6 && arg_arg_phase==1,AngleCmd(:)=single(0);
    | end
    | if arg_arg_angleReset,Centers(1:2)=AngleCmd;end
    | if arg_arg_reset,Centers(3)=YawCmd;end
    | if arg_arg_run && (arg_arg_phase==0 || arg_arg_phase==1) && uint8(arg_arg_controlMode)==0
    |  limit=single(30*pi/180);Angle=min(max(single(.5*pi*double(AngleCmd-Centers(1:2))),-limit),limit);
    | end
    | if arg_branch==6 && arg_arg_phase>=2,arg_arg_directRate(1)=arg_arg_flipRate;arg_arg_directRate(2)=single(0);end
    | if arg_branch==3,arg_arg_directRate(1)=single(0);end
    | if arg_arg_reset,arg_arg_directRate(:)=single(0);end
    | arg_arg_angle=Angle;
    | end
    | function y=rateCommand(x)
    | x=min(max(x,single(-1)),single(1));a=abs(x);t=a*(a*a*a*a*a*single(.5)+a*single(.5));
    | y=single(pi/180)*((single(1600)-single(70))*t+single(70)*a);if x<0,y=-y;end
    | end

== stateflow chart StampFly_StudentBlocks/Controllers/SelectRateReference ==
  state Calculate
    en: [rate]=stepFn(direct,rollPID,pitchPID,angleEnable);
    du: [rate]=stepFn(direct,rollPID,pitchPID,angleEnable);
  (default) -> Calculate
  data: direct function_input; rollPID function_input; pitchPID function_input; angleEnable function_input; rate function_output; direct input single; rollPID input single; pitchPID input single; angleEnable input boolean; rate output single
  function rate =stepFn(direct,rollPID,pitchPID,angleEnable):
    | function rate =stepFn(direct,rollPID,pitchPID,angleEnable)
    | % 日本語の説明はブロック注釈とDescriptionを参照。
    | %#codegen
    |             rate=direct;if angleEnable,rate(1)=rollPID;rate(2)=pitchPID;end
    | end

== stateflow chart StampFly_StudentBlocks/Controllers/SelectVerticalReference ==
  state Calculate
    en: [vRef]=stepFn(zRef,mode,auto,flipFlag);
    du: [vRef]=stepFn(zRef,mode,auto,flipFlag);
  (default) -> Calculate
  data: arg_zRef function_input; arg_mode function_input; arg_vRef function_output; arg_auto function_input; arg_flipFlag function_input; zRef input single; mode input uint8; vRef output single; auto input boolean; flipFlag input uint8
  function arg_vRef=stepFn(arg_zRef,arg_mode,arg_auto,arg_flipFlag):
    | function arg_vRef=stepFn(arg_zRef,arg_mode,arg_auto,arg_flipFlag)
    | % Auto高度補正が優先。公式else-ifの順序を維持。
    | %#codegen
    | arg_vRef=arg_zRef;if ~(arg_auto && arg_flipFlag==0) && arg_mode==5,arg_vRef=single(-.15);end
    | end

== stateflow chart StampFly_StudentBlocks/Controllers/ThrustCorrectionLimits ==
  note: 鉛直速度PID補正から推力を生成。10 msフィルター後、Auto高度では基準推力の0.85〜1.15倍に制限。
  state Calculate
    en: [thrust,filter,last]=stepFn(command,correction,base,auto,manual,velEnable,mode,dt,oldFilter,lastThrust,flipFlag);
    du: [thrust,filter,last]=stepFn(command,correction,base,auto,manual,velEnable,mode,dt,oldFilter,lastThrust,flipFlag);
  (default) -> Calculate
  data: arg_arg_command function_input; arg_arg_correction function_input; arg_arg_base function_input; arg_arg_auto function_input; arg_arg_manual function_input; arg_arg_velEnable function_input; arg_branch function_input; arg_arg_dt function_input; arg_arg_oldFilter function_input; arg_arg_lastThrust function_input; arg_arg_thrust function_output; arg_arg_filter function_output; arg_arg_last function_output; arg_arg_flipFlag function_input; command input single; correction input single; base input single; auto input boolean; manual input boolean; velEnable input boolean; mode input uint8; dt input single; oldFilter input single; lastThrust input single; thrust output single; filter output single; last output single; flipFlag input uint8
  function [arg_arg_thrust,arg_arg_filter,arg_arg_last]=stepFn(arg_arg_command,arg_arg_correction,arg_arg_base,arg_arg_auto,arg_arg_manual,arg_arg_velEnable,arg_branch,arg_arg_dt,arg_arg_oldFilter,arg_arg_lastThrust,arg_arg_flipFlag):
    | function [arg_arg_thrust,arg_arg_filter,arg_arg_last]=stepFn(arg_arg_command,arg_arg_correction,arg_arg_base,arg_arg_auto,arg_arg_manual,arg_arg_velEnable,arg_branch,arg_arg_dt,arg_arg_oldFilter,arg_arg_lastThrust,arg_arg_flipFlag)
    | % rate_control: Auto補正がLanding補正より優先。Flip中はAuto補正を停止。
    | %#codegen
    | arg_arg_thrust=arg_arg_command;arg_arg_filter=arg_arg_oldFilter;
    | if arg_branch==3,arg_arg_filter=single(0);elseif arg_arg_manual,arg_arg_filter=arg_arg_command;end
    | if arg_arg_velEnable
    |  arg_arg_filter=filterStep(single(double(arg_arg_base+arg_arg_correction)*3.7),arg_arg_dt,single(.01),arg_arg_filter);arg_arg_thrust=arg_arg_filter;
    |  if arg_arg_auto && arg_arg_flipFlag==0
    |   if double(arg_arg_thrust)/3.7>double(single(arg_arg_base*single(1.15))),arg_arg_thrust=single(3.7*double(arg_arg_base)*double(single(1.15)));end
    |   if double(arg_arg_thrust)/3.7<double(single(arg_arg_base*single(.85))),arg_arg_thrust=single(3.7*double(arg_arg_base)*double(single(.85)));end
    |  end
    | end
    | if arg_branch==3,arg_arg_thrust=arg_arg_lastThrust;arg_arg_last=arg_arg_lastThrust;else,arg_arg_last=arg_arg_thrust;end
    | end
    | function s=filterStep(u,h,T,s),s=s*T/(T+h)+u*h/(T+h);end
